simulink model "CorleyLorenz1998_HFI"  (R2024b)
settings: Solver=FixedStepDiscrete  StartTime=0  StopTime=1.1  FixedStep=TsHfi  RelTol=1e-3
InitFcn:
  | demoModel=bdroot; demoWorkspace=get_param(demoModel,'ModelWorkspace');
  | demoCases=getVariable(demoWorkspace,'DemoCases');
  | demoCaseName=get_param([demoModel '/Experiment_Settings'],'CaseName');
  | demoSelected=find(strcmp(demoCaseName,{demoCases.name}),1);
  | demoValues=demoCases(demoSelected).variables; demoNames=fieldnames(demoValues);
  | for demoIndex=1:numel(demoNames), assignin(demoWorkspace,demoNames{demoIndex},demoValues.(demoNames{demoIndex})); end
  | clear demoModel demoWorkspace demoCases demoCaseName demoSelected demoValues demoNames demoIndex;
model workspace (MAT data in the model file):
  BenchTheta = 1.04719758034
  DemoCases(1).name = 'standstill'
  DemoCases(1).variables.ScenarioData = [0 2.5e-05 5e-05 7.5e-05 0.0001 0.000125 0.00015 0.000175 0.0002 0.000225 0.00025 0.000275 ... (308007 elements, 44001x7)]
  DemoCases(1).variables.BenchTheta = 1.04719758034
  DemoCases(2).name = 'injection_off'
  DemoCases(2).variables.ScenarioData = [0 2.5e-05 5e-05 7.5e-05 0.0001 0.000125 0.00015 0.000175 0.0002 0.000225 0.00025 0.000275 ... (308007 elements, 44001x7)]
  DemoCases(2).variables.BenchTheta = 1.04719758034
  DemoCases(3).name = 'current_noise'
  DemoCases(3).variables.ScenarioData = [0 2.5e-05 5e-05 7.5e-05 0.0001 0.000125 0.00015 0.000175 0.0002 0.000225 0.00025 0.000275 ... (308007 elements, 44001x7)]
  DemoCases(3).variables.BenchTheta = 1.04719758034
  DemoCases(4).name = 'low_speed'
  DemoCases(4).variables.ScenarioData = [0 2.5e-05 5e-05 7.5e-05 0.0001 0.000125 0.00015 0.000175 0.0002 0.000225 0.00025 0.000275 ... (308007 elements, 44001x7)]
  DemoCases(4).variables.BenchTheta = 1.04719758034
  DemoCases(5).name = 'high_speed'
  DemoCases(5).variables.ScenarioData = [0 2.5e-05 5e-05 7.5e-05 0.0001 0.000125 0.00015 0.000175 0.0002 0.000225 0.00025 0.000275 ... (308007 elements, 44001x7)]
  DemoCases(5).variables.BenchTheta = 1.04719758034
  DemoCases(6).name = 'high_without_d_feedforward'
  DemoCases(6).variables.ScenarioData = [0 2.5e-05 5e-05 7.5e-05 0.0001 0.000125 0.00015 0.000175 0.0002 0.000225 0.00025 0.000275 ... (308007 elements, 44001x7)]
  DemoCases(6).variables.BenchTheta = 1.04719758034
  DemoCases(7).name = 'opposite_polarity'
  DemoCases(7).variables.ScenarioData = [0 2.5e-05 5e-05 7.5e-05 0.0001 0.000125 0.00015 0.000175 0.0002 0.000225 0.00025 0.000275 ... (308007 elements, 44001x7)]
  DemoCases(7).variables.BenchTheta = 3.57792496681
  RecordedSignalNames = {'ThetaTrue_rad'; 'OmegaTrue_radps'; 'ThetaElectrical_rad'; 'OmegaElectrical_radps'; 'InjectAlpha_V'; 'InjectBeta_V'; 'IDProjected_A'; 'IDCarrier_A'; 'Mixed_A'; 'AngleResidual'; 'CarrierReference'; 'IQProjected_A'; 'LoadTorqueEstimate_Nm'; 'IAlphaADC_A'; 'IBetaADC_A'; 'TorqueEstimate_Nm'; 'CarrierAmplitude_V'; 'DFeedforward'; 'ElectromagneticTorque_Nm'}
  ScenarioData = [0 2.5e-05 5e-05 7.5e-05 0.0001 0.000125 0.00015 0.000175 0.0002 0.000225 0.00025 0.000275 ... (308007 elements, 44001x7)]
values from neighbouring files (symbols this model uses):
  BpfA = 1.0 -1.60953951 0.692369938    [CorleyLorenz1998_HFI.sldd]
  BpfB = 0.153815016 0.0 -0.153815016    [CorleyLorenz1998_HFI.sldd]
  CarrierStep = 0.314159274    [CorleyLorenz1998_HFI.sldd]
  ErrorScale = 6.46270466    [CorleyLorenz1998_HFI.sldd]
  FluxPm = 0.013    [CorleyLorenz1998_HFI.sldd]
  Inertia = 0.0014    [CorleyLorenz1998_HFI.sldd]
  InvCarrierOmega = 7.95774686E-5    [CorleyLorenz1998_HFI.sldd]
  Ld = 0.00045    [CorleyLorenz1998_HFI.sldd]
  LpfA = 1.0 -0.959982038    [CorleyLorenz1998_HFI.sldd]
  LpfB = 0.0400179625    [CorleyLorenz1998_HFI.sldd]
  Lq = 0.0008    [CorleyLorenz1998_HFI.sldd]
  ObsL = 1446628.88    [CorleyLorenz1998_HFI.sldd]
  ObsP = 339.292    [CorleyLorenz1998_HFI.sldd]
  ObsV = 38373.0234    [CorleyLorenz1998_HFI.sldd]
  PolePairs = 2.0    [CorleyLorenz1998_HFI.sldd]
  Rstator = 0.24    [CorleyLorenz1998_HFI.sldd]
  ThetaHatInitial = 0.436332315    [CorleyLorenz1998_HFI.sldd]
  TsHfi = 2.5E-5    [CorleyLorenz1998_HFI.sldd]
  TsSingle = 2.5E-5    [CorleyLorenz1998_HFI.sldd]
  TwoPi = 6.28318548    [CorleyLorenz1998_HFI.sldd]
  Vdc = 48.0    [CorleyLorenz1998_HFI.sldd]
undefined symbols (not defined in the file or in its folder): DiscIntNeverNeededParam
(part 1 of 2)
settings Model: DataDictionary=CorleyLorenz1998_HFI.sldd  Creator=lxy  LastModifiedBy=lxy
settings DataIOCC: SaveTime=off

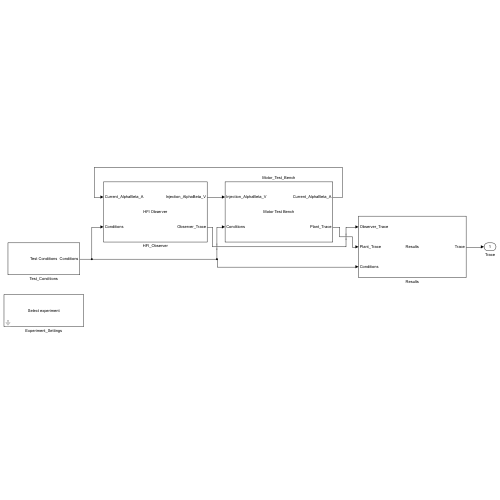
[thumbnail: Simulink's stored preview of the top-level diagram]
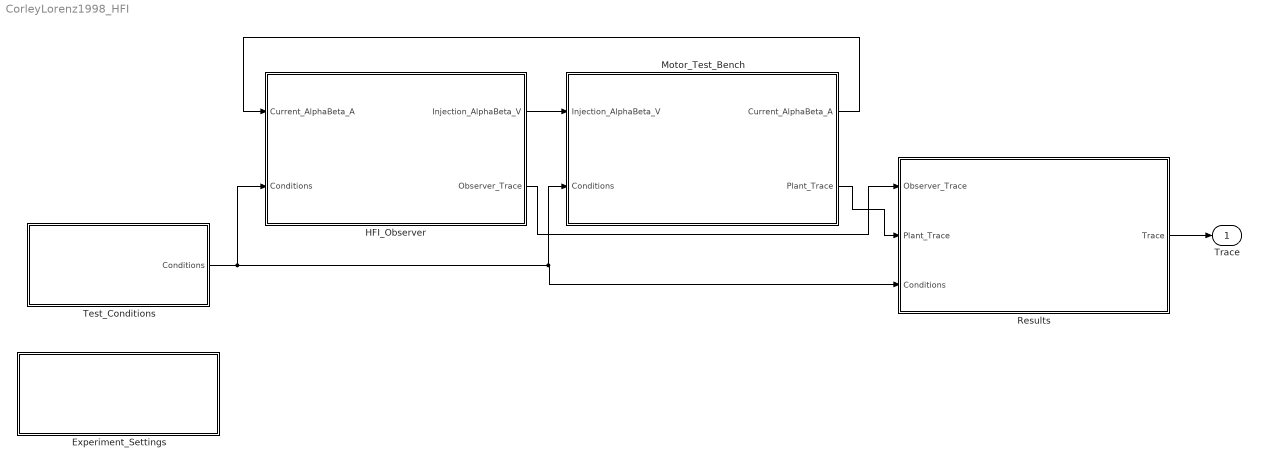
== system CorleyLorenz1998_HFI ==
  Experiment_Settings : Subsystem  mask{CaseName=low_speed}
      mask prompts: CaseName "Experiment"
      mask TypeOptions CaseName: standstill | injection_off | current_noise | low_speed | high_speed | high_without_d_feedforward | opposite_polarity
      mask Display: disp('Select experiment')
  HFI_Observer : Subsystem
      mask Display: disp('HFI Observer');port_label('input',1,'Current_AlphaBeta_A');port_label('input',2,'Conditions');port_label('output',1,'Injection_AlphaBeta_V');port_label('output',2,'Observer_Trace')
  Motor_Test_Bench : Subsystem
      mask Display: disp('Motor Test Bench');port_label('input',1,'Injection_AlphaBeta_V');port_label('input',2,'Conditions');port_label('output',1,'Current_AlphaBeta_A');port_label('output',2,'Plant_Trace')
  Results : Subsystem
      mask Display: disp('Results');port_label('input',1,'Observer_Trace');port_label('input',2,'Plant_Trace');port_label('input',3,'Conditions');port_label('output',1,'Trace')
  Test_Conditions : Subsystem
      mask Display: disp('Test Conditions');port_label('output',1,'Conditions')
  Trace : Outport
  wires:
  Results/1(Trace) -> Trace/1
  Test_Conditions/1(Conditions) -> Results/3(Conditions), Motor_Test_Bench/2(Conditions), HFI_Observer/2(Conditions)
  Motor_Test_Bench/1(Current_AlphaBeta_A) -> HFI_Observer/1(Current_AlphaBeta_A)
  HFI_Observer/1(Injection_AlphaBeta_V) -> Motor_Test_Bench/1(Injection_AlphaBeta_V)
  HFI_Observer/2(Observer_Trace) -> Results/1(Observer_Trace)
  Motor_Test_Bench/2(Plant_Trace) -> Results/2(Plant_Trace)
